simulink model "simLpvssCtTest"  (R2020a)
settings: Solver=VariableStepAuto  StartTime=0.0  StopTime=10.0  RelTol=1e-3
values from neighbouring files (symbols this model uses):
  P1 = lpvss(P1l)    [simulinkCoreTest.m]
  P1l = drss(nx,ny,nu);P1l.Ts = Ts    [simulinkCoreTest.m]
  P2 = lpvss(Ag,Bg,Cg,Dg,Ts)    [simulinkCoreTest.m]
  P3 = lpvlfr(Delta,G)    [simulinkCoreTest.m]
  x0 = randn(nx,1)    [simulinkCoreTest.m]
libraries: lpvcoreLibraryCore x3
settings Model: Creator=Patrick  LastModifiedBy=Patrick
settings DataIOCC: SaveOutput=off  SignalLogging=off  DSMLogging=off  SaveTime=off
settings DebuggingCC: AlgebraicLoopMsg=none

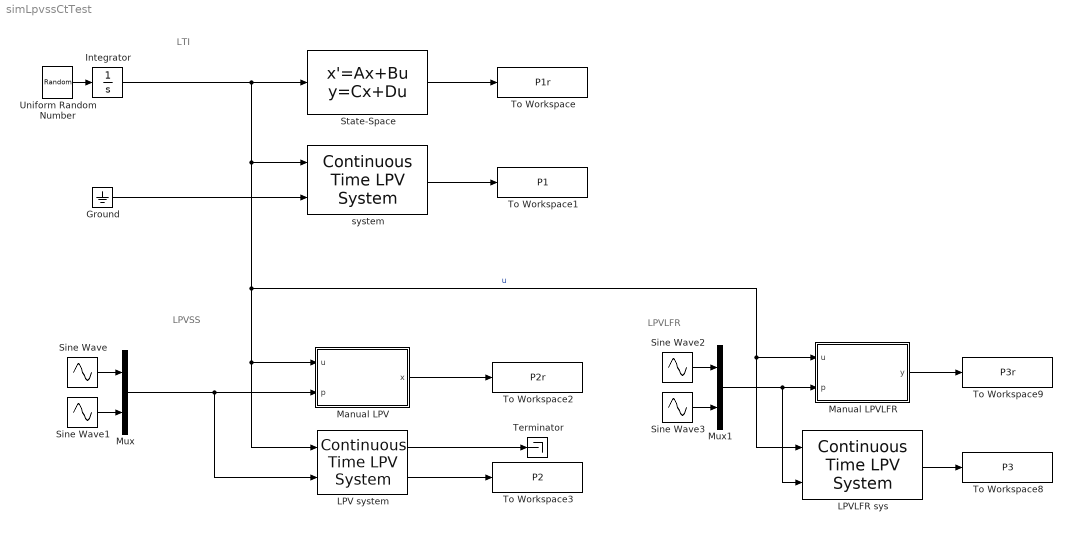
== system simLpvssCtTest ==
  note: LPVLFR
  note: LTI
  note: LPVSS
  Ground : Ground
  Integrator : Integrator
  LPV system : lpvcoreLibraryCore/Systems/Continuous Time LPV System  P=P2  x0=0  stateOut=on
      settings: SourceProductName=LPVcore
  LPVLFR sys : lpvcoreLibraryCore/Systems/Continuous Time LPV System  P=P3  x0=0  stateOut=off
      settings: SourceProductName=LPVcore
  Manual LPV : Subsystem
  Manual LPVLFR : Subsystem
  Mux : Mux  Inputs=2
  Mux1 : Mux  Inputs=2
  Sine Wave : Sin  Bias=1  SampleTime=0
  Sine Wave1 : Sin  Bias=1  Frequency=2  SampleTime=0
  Sine Wave2 : Sin  Amplitude=.2  SampleTime=0
  Sine Wave3 : Sin  Amplitude=.2  Frequency=2  SampleTime=0
  State-Space : StateSpace  A=P1l.A  B=P1l.B  C=P1l.C  D=P1l.D  InitialCondition=x0
  Terminator : Terminator
  To Workspace : ToWorkspace  VariableName=P1r  SampleTime=-1
  To Workspace1 : ToWorkspace  VariableName=P1  SampleTime=-1
  To Workspace2 : ToWorkspace  VariableName=P2r  SampleTime=-1
  To Workspace3 : ToWorkspace  VariableName=P2  SampleTime=-1
  To Workspace8 : ToWorkspace  VariableName=P3  SampleTime=-1
  To Workspace9 : ToWorkspace  VariableName=P3r  SampleTime=-1
  Uniform Random Number : UniformRandomNumber  SampleTime=0.1
  system : lpvcoreLibraryCore/Systems/Continuous Time LPV System  P=P1  x0=x0  stateOut=off
      settings: SourceProductName=LPVcore
  wires:
  Ground/1 -> system/2
  Uniform Random Number/1 -> Integrator/1
  Manual LPV/1(x) -> To Workspace2/1
  system/1 -> To Workspace1/1
  State-Space/1 -> To Workspace/1
  Sine Wave/1 -> Mux/1
  Sine Wave1/1 -> Mux/2
  Integrator/1 -> State-Space/1, system/1, Manual LPVLFR/1(u), LPVLFR sys/1, LPV system/1, Manual LPV/1(u)  "u"
  Mux/1 -> LPV system/2, Manual LPV/2(p)
  Sine Wave3/1 -> Mux1/2
  Sine Wave2/1 -> Mux1/1
  Mux1/1 -> LPVLFR sys/2, Manual LPVLFR/2(p)
  LPVLFR sys/1 -> To Workspace8/1
  Manual LPVLFR/1(y) -> To Workspace9/1
  LPV system/2 -> To Workspace3/1
  LPV system/1 -> Terminator/1

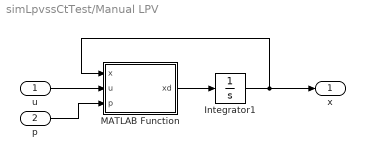
== system simLpvssCtTest/Manual LPV ==
  u : Inport
  p : Inport  Port=2
  Integrator1 : Integrator  InitialCondition=[0;0]
  MATLAB Function : MATLAB Function  TreatAsAtomicUnit=on
  x : Outport
  wires:
  u/1 -> MATLAB Function/2(u)
  MATLAB Function/1(xd) -> Integrator1/1
  Integrator1/1 -> x/1, MATLAB Function/1(x)
  p/1 -> MATLAB Function/3(p)

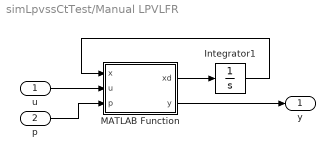
== system simLpvssCtTest/Manual LPVLFR ==
  u : Inport
  p : Inport  Port=2
  Integrator1 : Integrator  InitialCondition=[0;0]
  MATLAB Function : MATLAB Function  TreatAsAtomicUnit=on
  y : Outport
  wires:
  u/1 -> MATLAB Function/2(u)
  MATLAB Function/1(xd) -> Integrator1/1
  Integrator1/1 -> MATLAB Function/1(x)
  p/1 -> MATLAB Function/3(p)
  MATLAB Function/2(y) -> y/1

== matlab function simLpvssCtTest/Manual LPVLFR/MATLAB Function ==
  data: x input size=2; u input; xd output size=2; p input; y output
function [xd,y] = fcn(x,u,p)
A0 = diag([-1 -2]);
Bw = [1 3;2 6];
Bu = [1;1];
Cz = [1 3];
Cy = [2 1];
Dzw = [-1 -1];
Dzu = 3;
Dyw = [2 3];
Dyu = 5;
Delta = @(p1,p2) [p1;p2];
Deltap = Delta(p(1),p(2));
Mid = Deltap/(1-Dzw*Deltap);

A = A0+Bw*Mid*Cz;
B = Bu+Bw*Mid*Dzu;
C = Cy+Dyw*Mid*Cz;
D = Dyu+Dyw*Mid*Dzu;

xd = A*x+B*u;
y = C*x+D*u;

== matlab function simLpvssCtTest/Manual LPV/MATLAB Function ==
  data: x input size=2; u input; xd output size=2; p input
function xd = fcn(x,u,p)
xd = zeros(2,1);
xd(1) = x(2);
xd(2) = -x(1)-20*p(1)*x(1)-p(2)^2*x(2)+u;
